simulink model "UAV_GuidanceWaypointFollowing"  (R2026a)
settings: Solver=ode45  StopTime=60  MaxStep=0.01
model workspace (MAT data in the model file):
  ctrl.mass = 0.1
  ctrl.g = 9.81
  ctrl.Kp_pos = 0.8
  ctrl.vMaxXY = 3
  ctrl.vMaxZ = 1.5
  ctrl.Kv = 2
  ctrl.tiltMax = 0.35
  ctrl.thrustMax = 2
  ctrl.Kyaw = 2
  ctrl.yawRateMax = 1
  gravityNED = 9.81
  hoverThrust = 0.981
  lookaheadDist = 3
  transitionRadius = 1.5
  uavMass = 0.1
  waypoints = [0  0  -5; 20  0  -5; 20  20  -5; 0  20  -5; 0  0  -5]
libraries: uavalgslib x2, uavutilslib x1
settings Model: Creator=PattarapolSangaroon  LastModifiedBy=PattarapolSangaroon

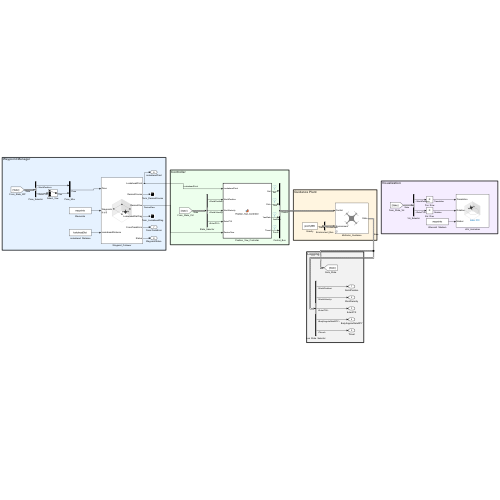
[thumbnail: Simulink's stored preview of the top-level diagram]
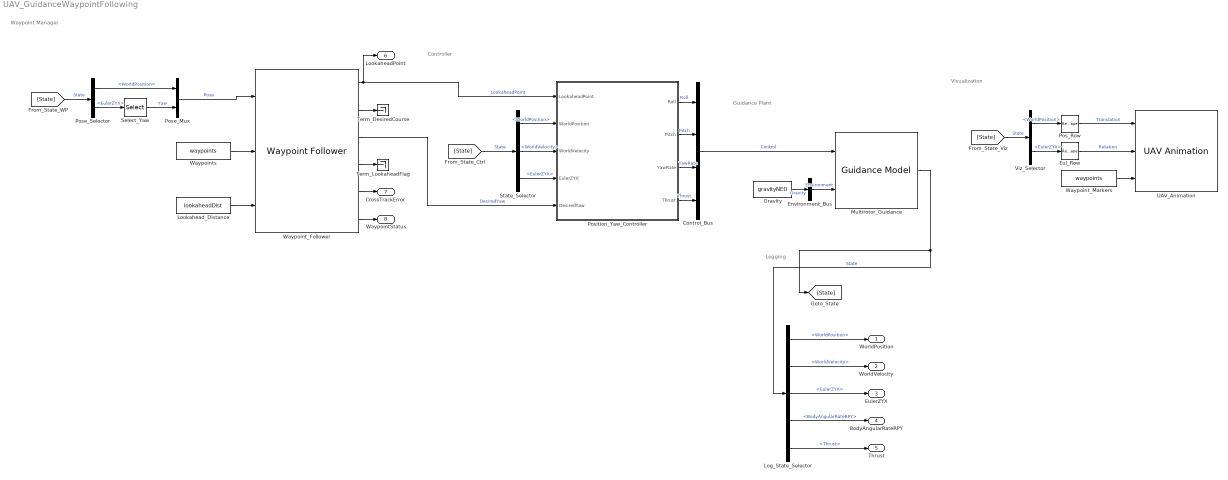
== system UAV_GuidanceWaypointFollowing ==
  note: Waypoint Manager
  note: Controller
  note: Guidance Plant
  note: Visualization
  note: Logging
  Control_Bus : BusCreator  Inputs=4  OutDataTypeStr=Bus: MultirotorGuidanceControlBus  NonVirtualBus=on
  Environment_Bus : BusCreator  Inputs=1  OutDataTypeStr=Bus: MultirotorGuidanceEnvironmentBus  NonVirtualBus=on
  Eul_Row : Reshape  OutputDimensionality=Customize  OutputDimensions=[1 3]
  Gravity : Constant  Value=gravityNED
  Log_State_Selector : BusSelector  OutputSignals=WorldPosition,WorldVelocity,EulerZYX,BodyAngularRateRPY,Thrust
  Lookahead_Distance : Constant  Value=lookaheadDist
  Multirotor_Guidance : uavalgslib/Guidance Model  ModelType=MultirotorGuidance  NumInstances=1  SpecifiedDataType=double  SimulateUsing=Code generation  InitialWorldPositionMultirotor=[0; 0; 0]  InitialWorldVelocityMultirotor=[0; 0; 0]  InitialEulerZYXMultirotor=[0; 0; 0]  InitialBodyAngularRateRPYMultirotor=[0; 0; 0]  InitialThrustMultirotor=hoverThrust  InitialNorthFixedWing=0  InitialEastFixedWing=0  InitialHeightFixedWing=0  InitialAirSpeedFixedWing=0  InitialHeadingAngleFixedWing=0  InitialFlightPathAngleFixedWing=0  InitialRollAngleFixedWing=0  InitialRollAngleRateFixedWing=0  PDRollMultirotor=[3402.97,116.67]  PDPitchMultirotor=[3402.97, 116.67]  PYawRateMultirotor=1950  PThrustMultirotor=3900  MassMultirotor=uavMass  PHeightFixedWing=3.9  PHeadingAngleFixedWing=3.9  PFlightPathAngleFixedWing=39  PDRollFixedWing=[3402.97, 116.67]  PAirSpeedFixedWing=1  FlightPathAngleLimitsFixedWing=[-pi/2, pi/2]  StateBusName='MultirotorGuidanceStateBus'  ControlBusName='MultirotorGuidanceControlBus'  EnvironmentBusName='MultirotorGuidanceEnvironmentBus'  DataType=double
  Pos_Row : Reshape  OutputDimensionality=Customize  OutputDimensions=[1 3]
  Pose_Mux : Mux  Inputs=2
  Pose_Selector : BusSelector  OutputSignals=WorldPosition,EulerZYX
  Position_Yaw_Controller : MATLAB Function  TreatAsAtomicUnit=on
  Select_Yaw : Selector  InputPortWidth=3  IndexOptions=Index vector (dialog)  Indices=1  OutputSizes=1
  State_Selector : BusSelector  OutputSignals=WorldPosition,WorldVelocity,EulerZYX
  Term_DesiredCourse : Terminator
  Term_LookaheadFlag : Terminator
  UAV_Animation : uavutilslib/UAV Animation  NumUAV=1  DynamicUAVConfig=off  UAVType=Multirotor  UAVSize=1  UAVColor=[1 0 0]  UAVTrajectoryAlpha=1  AlwaysShowAnimation=on  AxisLimits=[-Inf Inf;-Inf Inf;-Inf Inf]  TrajectoryBufferSize=100000  InertialZDirection=Down  RotationFormat=Euler ZYX  DrawMarkers=on  SampleTime=0.1
  Viz_Selector : BusSelector  OutputSignals=WorldPosition,EulerZYX
  Waypoint_Follower : uavalgslib/Waypoint Follower  UAVType=multirotor  StartFrom=first  TransitionRadiusSource=internal  TransitionRadius=transitionRadius  MinLookaheadDistance=0.1  HoverAtLastWaypoint=on  InterpolateYaw=on  YawInput=off  ShowCrossTrackErrorOutput=on  ShowStatusOutput=on  ShowWaypointIndexOutput=off  SimulateUsing=Code generation
  Waypoint_Markers : Constant  Value=waypoints
  Waypoints : Constant  Value=waypoints
  WorldPosition : Outport
  WorldVelocity : Outport  Port=2
  EulerZYX : Outport  Port=3
  BodyAngularRateRPY : Outport  Port=4
  Thrust : Outport  Port=5
  LookaheadPoint : Outport  Port=6
  CrossTrackError : Outport  Port=7
  WaypointStatus : Outport  Port=8
  wires:
  [State] -> Viz_Selector/1  "State"
  Viz_Selector/1 -> Pos_Row/1  "<WorldPosition>"
  Waypoint_Markers/1 -> UAV_Animation/3
  Viz_Selector/2 -> Eul_Row/1  "<EulerZYX>"
  Eul_Row/1 -> UAV_Animation/2  "Rotation"
  Pos_Row/1 -> UAV_Animation/1  "Translation"
  Environment_Bus/1 -> Multirotor_Guidance/2  "Environment"
  Gravity/1 -> Environment_Bus/1  "Gravity"
  Multirotor_Guidance/1 -> Log_State_Selector/1, [State]  "State"
  Control_Bus/1 -> Multirotor_Guidance/1  "Control"
  [State] -> State_Selector/1  "State"
  State_Selector/3 -> Position_Yaw_Controller/4(EulerZYX)  "<EulerZYX>"
  State_Selector/2 -> Position_Yaw_Controller/3(WorldVelocity)  "<WorldVelocity>"
  State_Selector/1 -> Position_Yaw_Controller/2(WorldPosition)  "<WorldPosition>"
  Position_Yaw_Controller/3(YawRate) -> Control_Bus/3  "YawRate"
  Position_Yaw_Controller/2(Pitch) -> Control_Bus/2  "Pitch"
  Position_Yaw_Controller/1(Roll) -> Control_Bus/1  "Roll"
  Position_Yaw_Controller/4(Thrust) -> Control_Bus/4  "Thrust"
  Waypoint_Follower/3 -> Position_Yaw_Controller/5(DesiredYaw)  "DesiredYaw"
  [State] -> Pose_Selector/1  "State"
  Pose_Selector/1 -> Pose_Mux/1  "<WorldPosition>"
  Lookahead_Distance/1 -> Waypoint_Follower/3
  Pose_Mux/1 -> Waypoint_Follower/1  "Pose"
  Pose_Selector/2 -> Select_Yaw/1  "<EulerZYX>"
  Select_Yaw/1 -> Pose_Mux/2  "Yaw"
  Waypoint_Follower/1 -> Position_Yaw_Controller/1(LookaheadPoint), LookaheadPoint/1  "LookaheadPoint"
  Waypoints/1 -> Waypoint_Follower/2
  Waypoint_Follower/2 -> Term_DesiredCourse/1
  Waypoint_Follower/4 -> Term_LookaheadFlag/1
  Waypoint_Follower/5 -> CrossTrackError/1
  Waypoint_Follower/6 -> WaypointStatus/1
  Log_State_Selector/1 -> WorldPosition/1  "<WorldPosition>"
  Log_State_Selector/2 -> WorldVelocity/1  "<WorldVelocity>"
  Log_State_Selector/3 -> EulerZYX/1  "<EulerZYX>"
  Log_State_Selector/4 -> BodyAngularRateRPY/1  "<BodyAngularRateRPY>"
  Log_State_Selector/5 -> Thrust/1  "<Thrust>"

== matlab function UAV_GuidanceWaypointFollowing/Position_Yaw_Controller ==
  data: LookaheadPoint input; Roll output; WorldPosition input; WorldVelocity input; EulerZYX input; DesiredYaw input; Pitch output; YawRate output; Thrust output; ctrl parameter
function [Roll, Pitch, YawRate, Thrust] = Position_Yaw_Controller(LookaheadPoint, WorldPosition, WorldVelocity, EulerZYX, DesiredYaw, ctrl)
%#codegen
% Waypoint tracking controller for the multirotor Guidance Model.
% Source of the MATLAB Function block in UAV_GuidanceWaypointFollowing.slx.
% Frame: NED [north east down]. EulerZYX = [yaw pitch roll].
% Small-angle Guidance Model kinematics (consistent with the step tests:
% +roll -> +east, +pitch -> -north):
%   aN = -g*(pitch*cos(yaw) + roll*sin(yaw))
%   aE = -g*(pitch*sin(yaw) - roll*cos(yaw))
%   aD =  g - Thrust*cos(roll)*cos(pitch)/mass

yaw = EulerZYX(1);

% Outer loop: position error -> velocity command (with limits)
vCmd = ctrl.Kp_pos * (LookaheadPoint(:) - WorldPosition(:));
speedXY = norm(vCmd(1:2));
if speedXY > ctrl.vMaxXY
    vCmd(1:2) = vCmd(1:2) * (ctrl.vMaxXY / speedXY);
end
vCmd(3) = min(max(vCmd(3), -ctrl.vMaxZ), ctrl.vMaxZ);

% Inner loop: velocity error -> acceleration command (NED)
aCmd = ctrl.Kv * (vCmd - WorldVelocity(:));

% Rotate horizontal acceleration into the heading frame
aFwd   =  cos(yaw)*aCmd(1) + sin(yaw)*aCmd(2);
aRight = -sin(yaw)*aCmd(1) + cos(yaw)*aCmd(2);

% Acceleration -> attitude and thrust
Pitch = min(max(-aFwd   / ctrl.g, -ctrl.tiltMax), ctrl.tiltMax);
Roll  = min(max( aRight / ctrl.g, -ctrl.tiltMax), ctrl.tiltMax);
Thrust = ctrl.mass * (ctrl.g - aCmd(3)) / (cos(Roll) * cos(Pitch));
Thrust = min(max(Thrust, 0), ctrl.thrustMax);

% Yaw: wrapped heading error -> yaw-rate command
yawErr = atan2(sin(DesiredYaw - yaw), cos(DesiredYaw - yaw));
YawRate = min(max(ctrl.Kyaw * yawErr, -ctrl.yawRateMax), ctrl.yawRateMax);
end
